simulink model "RM3_R2020b"  (R2020b)
settings: Solver=ode4  StartTime=0  StopTime=400  FixedStep=0.1  MaxStep=0.1  RelTol=1e-3  EnableMultiTasking=on
values from neighbouring files (symbols this model uses):
  F_ext_b1 = testCase.loadUserDefinedForce()    [TestRM3UserDefinedForce.m]    (also in wecSimInputFile.m = [0,0,5.0e5,0,0,0])
  simu = simulationClass()    [wecSimInputFile.m]
undefined symbols (not defined in the file or in its folder): body, constraint, pto, X, Y, Z
libraries: sm_lib x3, WECSim_Lib_Body_Elements x2, nesl_utility x2, WECSim_Lib_Constraints x1, WECSim_Lib_Frames x1, simulink x1, WECSim_Lib_PTOs x1
settings Model: Creator=mlawson  LastModifiedBy=rsaucie
settings SolverCC: ZeroCrossControl=DisableAll  AlgebraicLoopSolver=LineSearch  AutoInsertRateTranBlk=on
settings DataIOCC: SaveFormat=Array  SaveOutput=off  SaveTime=off  ReturnWorkspaceOutputs=off
settings OptimizationCC: LifeSpan=inf  SimCompilerOptimization=on
settings DebuggingCC: MergeDetectMultiDrivingBlocksExec=none  SolverPrmCheckMsg=warning  AllowSymbolicDim=off  StateNameClashWarn=warning  SFUnexpectedBacktrackingDiag=warning  SFNoUnconditionalDefaultTransitionDiag=warning  SFExecutionAtInitializationDiag=none  ArithmeticOperatorsInVariantConditions=warning
settings HardwareCC: ProdBitPerPointer=32  ProdBitPerSizeT=32  ProdBitPerPtrDiffT=32  ProdLargestAtomicFloat=None  ProdIntDivRoundTo=Undefined  ProdEndianess=Unspecified  ProdWordSize=32  ProdHWDeviceType=32-bit Generic
settings ModelReferenceCC: PropagateSignalLabelsOutOfModel=off
settings SFSimCC: SimUseLocalCustomCode=off  CustomCodeUndefinedFunction=UseInterfaceOnly
settings RTWCC: RTWUseLocalCustomCode=off
settings CodeAppCC: StateflowObjectComments=on
settings GRTTargetCC: TargetLangStandard=C89/C90 (ANSI)
settings ConfigComp: CovMetricSettings=dw  CovSaveCumulativeToWorkspaceVar=on  CovSaveSingleToWorkspaceVar=on  CovExternalEMLEnable=off  CovSFcnEnable=off  CovBoundaryAbsTol=1.0e-5
settings SimscapeCC: SimscapeNormalizeSystem=off
settings ConfigurationSet: Description=SimMechanics 2G
settings ExplorerConfigSet: SimMechanicsOpenEditorOnUpdate=off  InternalSimMechanicsExplorerSettings="<ExplorerConfiguration><canonicalview>default</canonicalview><TilePanel><TileInfo><Tiles Columns=\"1\" Count=\"1\" Rows=\"1\"><Column Left=\"2\" Weight=\"1\"/><Column Left=\"1335\"/><Row Top=\"2\" Weight=\"1\"/><Row Top=\"911\"/><Tile Height=\"1\" Width=\"1\" X=\"0\" Y=\"0\"/></Tiles></TileInfo><SceneInfo><SceneViewer><BGColor><R>0.60000002384185791</R><G>0.60000002384185791</G><B>0.60000002384185791</B></BGColor><Camera><Position><X>365.37645888990272</X><Y>-369.82486814446582</Y><Z>359.64809521743916</Z></Position><Center><X>-6.7351450971904585</X><Y>2.2867358426280204</Y><Z>-12.463508769654169</Z></Center><Up><X>-0.40824829046386307</X><Y>0.40824829046386307</Y><Z>0.81649658092772615</Z></Up><Left>-57.820127362122818</Left><Right>57.820127362122818</Right><Bottom>-38.308817187253304</Bottom><Top>38.308817187253304</Top></Camera></SceneViewer></SceneInfo></TilePanel></ExplorerConfiguration>"

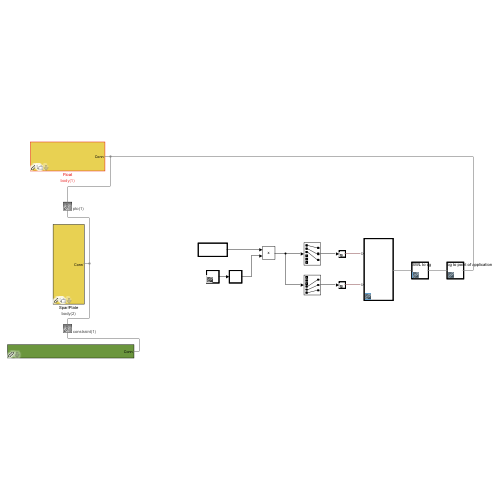
[thumbnail: Simulink's stored preview of the top-level diagram]
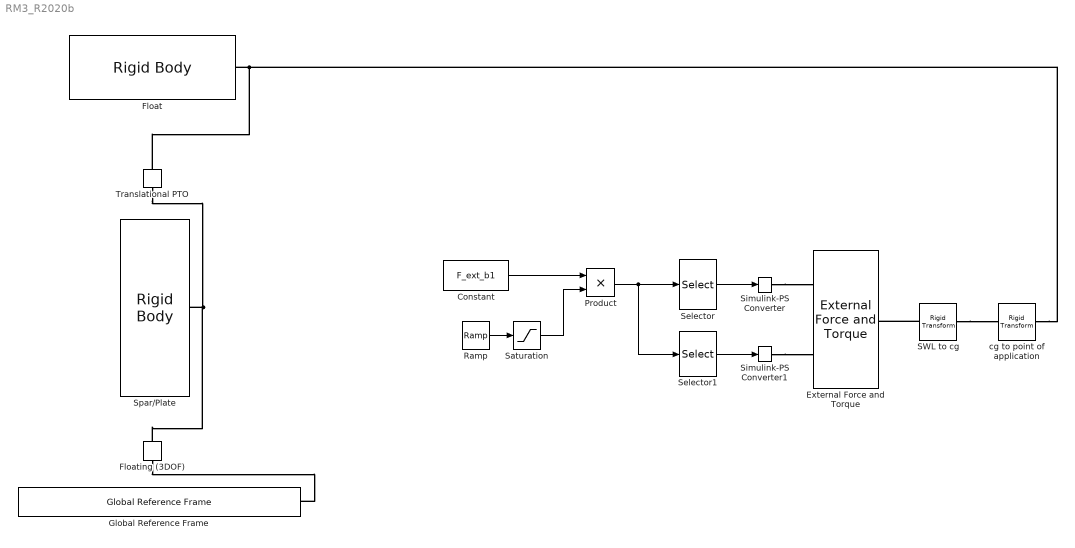
== system RM3_R2020b ==
  Constant : Constant  Value=F_ext_b1
  External Force and Torque : sm_lib/Forces and Torques/External Force and Torque  EnableForceX=off  EnableForceY=off  EnableForceZ=off  EnableForce=on  ForceResolutionFrame=AttachedFrame  EnableTorqueX=off  EnableTorqueY=off  EnableTorqueZ=off  EnableTorque=on  TorqueResolutionFrame=AttachedFrame
  Float : WECSim_Lib_Body_Elements/Rigid Body  body=body(1)
  Floating (3DOF) : WECSim_Lib_Constraints/Floating (3DOF)  constraint=constraint(1)
      settings: AttributesFormatString=%<constraint>  SourceProductName=WEC-Sim
  Global Reference Frame : WECSim_Lib_Frames/Global Reference Frame  waves=waves  simu=simu
      settings: SourceProductName=WEC-Sim
  Product : Product
  Ramp : simulink/Sources/Ramp  slope=1/(simu.rampTime)  start=0  InitialOutput=0
  SWL to cg : sm_lib/Frames and Transforms/Rigid Transform  RotationMethod=None  FollAlignAxisA=+X  BaseAlignAxisA=+Y  FollAlignAxisB=+Y  BaseAlignAxisB=+Z  RotationStandardAxis=+Z  RotationAngle=0  RotationAngleUnits=deg  RotationArbitraryAxis=[0 0 1]  RotationSequenceAxes=FollowerAxes  RotationSequence=XYX  RotationSequenceAngles=[0 0 0]  RotationSequenceAnglesUnits=deg  RotationMatrix=[1 0 0;0 1 0;0 0 1]  Quaternion=[1 0 0 0]  TranslationMethod=Cartesian  TranslationCartesianOffset=body(1).centerGravity  TranslationCartesianOffsetUnits=m  TranslationStandardAxis=+Z  TranslationStandardOffset=0  TranslationStandardOffsetUnits=m  TranslationROffset=0  TranslationROffsetUnits=m  TranslationThetaOffset=0  TranslationThetaOffsetUnits=deg  TranslationZOffset=0  TranslationZOffsetUnits=m
  Saturation : Saturate  UpperLimit=1  LowerLimit=0
  Selector : Selector  InputPortWidth=6  IndexOptions=Index vector (dialog)  Indices=[1:3]  OutputSizes=1
  Selector1 : Selector  InputPortWidth=6  IndexOptions=Index vector (dialog)  Indices=[4:6]  OutputSizes=1
  Simulink-PS Converter : nesl_utility/Simulink-PS Converter  PhysicalDomain=network_engine_domain  SubClassName=ps_input  LeftPortType=input  RightPortType=output  PseudoPeriodic=off  Frequencies=[]  NoiseDistribution=none  NoiseParameters=[]  Unit=1  AffineConversion=off  FilteringAndDerivatives=provide  SimscapeFilterOrder=1  InputFilterTimeConstant=0.001  UdotUserProvided=0
  Simulink-PS Converter1 : nesl_utility/Simulink-PS Converter  PhysicalDomain=network_engine_domain  SubClassName=ps_input  LeftPortType=input  RightPortType=output  PseudoPeriodic=off  Frequencies=[]  NoiseDistribution=none  NoiseParameters=[]  Unit=1  AffineConversion=off  FilteringAndDerivatives=provide  SimscapeFilterOrder=1  InputFilterTimeConstant=0.001  UdotUserProvided=0
  Spar/Plate : WECSim_Lib_Body_Elements/Rigid Body  body=body(2)
  Translational PTO : WECSim_Lib_PTOs/Translational PTO  pto=pto(1)
      settings: AttributesFormatString=%<pto>  SourceProductName=WEC-Sim
  cg to point of application : sm_lib/Frames and Transforms/Rigid Transform  RotationMethod=None  FollAlignAxisA=+X  BaseAlignAxisA=+Y  FollAlignAxisB=+Y  BaseAlignAxisB=+Z  RotationStandardAxis=+Z  RotationAngle=0  RotationAngleUnits=deg  RotationArbitraryAxis=[0 0 1]  RotationSequenceAxes=FollowerAxes  RotationSequence=XYX  RotationSequenceAngles=[0 0 0]  RotationSequenceAnglesUnits=deg  RotationMatrix=[1 0 0;0 1 0;0 0 1]  Quaternion=[1 0 0 0]  TranslationMethod=Cartesian  TranslationCartesianOffset=[10 0 0]  TranslationCartesianOffsetUnits=m  TranslationStandardAxis=+Z  TranslationStandardOffset=0  TranslationStandardOffsetUnits=m  TranslationROffset=0  TranslationROffsetUnits=m  TranslationThetaOffset=0  TranslationThetaOffsetUnits=deg  TranslationZOffset=0  TranslationZOffsetUnits=m
  wires:
  Selector/1 -> Simulink-PS Converter/1
  Selector1/1 -> Simulink-PS Converter1/1
  Ramp/1 -> Saturation/1
  Constant/1 -> Product/1
  Saturation/1 -> Product/2
  Product/1 -> Selector1/1, Selector/1
  connections:
  Floating (3DOF)/LConn1 -- Global Reference Frame/RConn1
  Spar/Plate/RConn1 -- Floating (3DOF)/RConn1 -- Translational PTO/RConn1
  Translational PTO/LConn1 -- cg to point of application/RConn1 -- Float/RConn1
  SWL to cg/LConn1 -- External Force and Torque/RConn1
  SWL to cg/RConn1 -- cg to point of application/LConn1
  Simulink-PS Converter/RConn1 -- External Force and Torque/LConn1
  Simulink-PS Converter1/RConn1 -- External Force and Torque/LConn2
